simulink model "Earthquake_Damped"  (R2026a)
settings: Solver=VariableStepAuto  StopTime=20

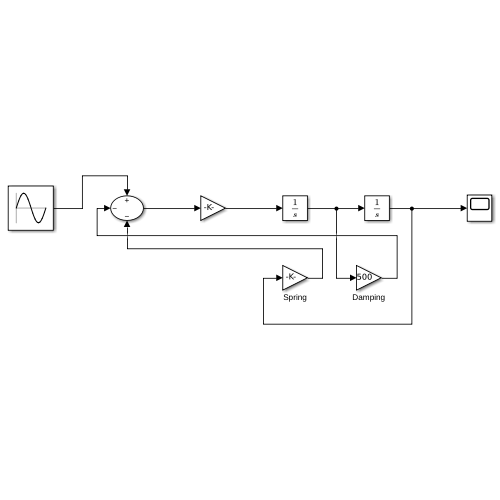
[thumbnail: Simulink's stored preview of the top-level diagram]
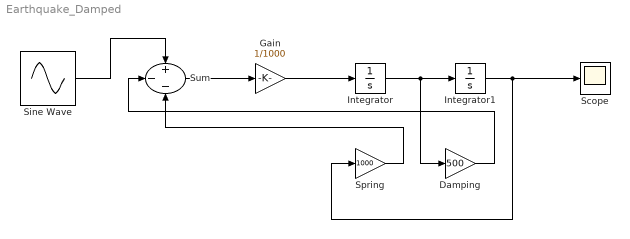
== system Earthquake_Damped ==
  Damping : Gain  Gain=500
  Gain : Gain  Gain=1/1000
  Integrator : Integrator
  Integrator1 : Integrator
  Scope : Scope
      settings: ActiveDisplayYMinimum=-1.0684506140163186  ActiveDisplayYMaximum=6.1088110507421032
  Sine Wave : Sin  Amplitude=1000  Frequency=3  SampleTime=0
  Spring : Gain  Gain=1000
  Sum : Sum  Inputs=+--
  wires:
  Sine Wave/1 -> Sum/1
  Sum/1 -> Gain/1
  Gain/1 -> Integrator/1
  Integrator/1 -> Integrator1/1, Damping/1
  Integrator1/1 -> Spring/1, Scope/1
  Spring/1 -> Sum/3
  Damping/1 -> Sum/2
